simulink model "Plotter_Data"  (R2024a)
settings: Solver=ode3  StartTime=0.0  StopTime=100  FixedStep=0.01  RelTol=1e-3
values from neighbouring files (symbols this model uses):
  n = 30    [CacFunctionTrongSimulink_LQR.m]
undefined symbols (not defined in the file or in its folder): LF
libraries: amg_usbconverter_n_connect_lib x2
settings Model: Creator=nguye  LastModifiedBy=nguye

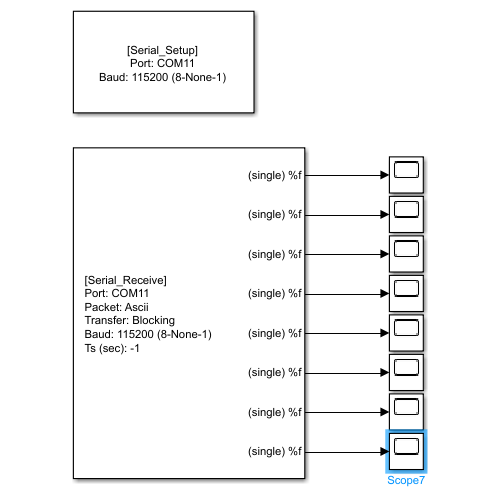
[thumbnail: Simulink's stored preview of the top-level diagram]
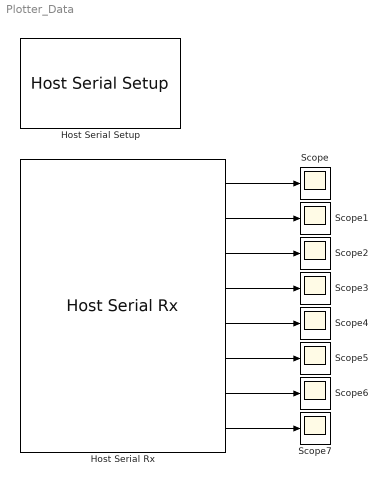
== system Plotter_Data ==
  Host Serial Rx : amg_usbconverter_n_connect_lib/Host Serial Rx  conf=rx  port=COM11  baudrate=115200  databits=8  parity=None  stopbit=1  flowcontrol=None  transfer=Blocking  timeout=5  packetmode=Ascii  enableinitialvalues=off  initialvalues=[]  binheader='7E 7E'  binterminator='03 03'  porttype_double=0  porttype_single=0  porttype_int8=0  porttype_uint8=0  porttype_int16=0  porttype_uint16=0  porttype_int32=0  porttype_uint32=2  asciiformat='%f,%f,%f,%f,%f,%f,%f,%f'  rx_asciiterminator="LF (0x0A - \"\\n\")"  tx_asciiterminator="CRLF (0x0D 0x0A - \"\\r\\n\")"  sampletime=0.02  enablecustomportlabel=off  cinputportlabel=0  coutputportlabel=A  portpinstr=0  blockid=HostSerialRx  inputporttype=[]  inputportwidth=[]  inputportlabel={}  outputporttype=[1 1 1 1 1 1 1 1]  outputportwidth=[1 1 1 1 1 1 1 1]  outputportlabel={'(single) %f','(single) %f','(single) %f','(single) %f','(single) %f','(single) %f','(single) %f','(single) %f'}  compat=0  optionstring=[]  autoport='COM11'
  Host Serial Setup : amg_usbconverter_n_connect_lib/Host Serial Setup  conf=setup  port=COM11  baudrate=115200  databits=8  parity=None  stopbit=1  flowcontrol=None  transfer=Blocking  timeout=2  packetmode=Binary  initialvalues=[]  binheader='7E 7E'  binterminator='03 03'  porttype_double=0  porttype_single=1  porttype_int8=0  porttype_uint8=0  porttype_int16=0  porttype_uint16=0  porttype_int32=0  porttype_uint32=2  asciiformat='%d %u %x'  rx_asciiterminator="CRLF (0x0D 0x0A - \"\\r\\n\")"  tx_asciiterminator="CRLF (0x0D 0x0A - \"\\r\\n\")"  sampletime=0.01  enablecustomportlabel=off  cinputportlabel=0  coutputportlabel=A  portpinstr=0  blockid=HostSerialSetup  inputporttype=[]  inputportwidth=[]  inputportlabel={}  outputporttype=[]  outputportwidth=[]  outputportlabel={}  compat=0  optionstring=[]  autoport='COM11'
  Scope{,1..7} (8 alike) : Scope
  wires:
  Host Serial Rx/1 -> Scope/1
  Host Serial Rx/2 -> Scope1/1
  Host Serial Rx/3 -> Scope2/1
  Host Serial Rx/4 -> Scope3/1
  Host Serial Rx/5 -> Scope4/1
  Host Serial Rx/6 -> Scope5/1
  Host Serial Rx/7 -> Scope6/1
  Host Serial Rx/8 -> Scope7/1
